simulink model "drive_fb_pack"  (R2026b)
settings: Solver=VariableStepAuto
undefined symbols (not defined in the file or in its folder): P
libraries: svdutilitieslib x3
settings Model: Creator=aomar  LastModifiedBy=aomar

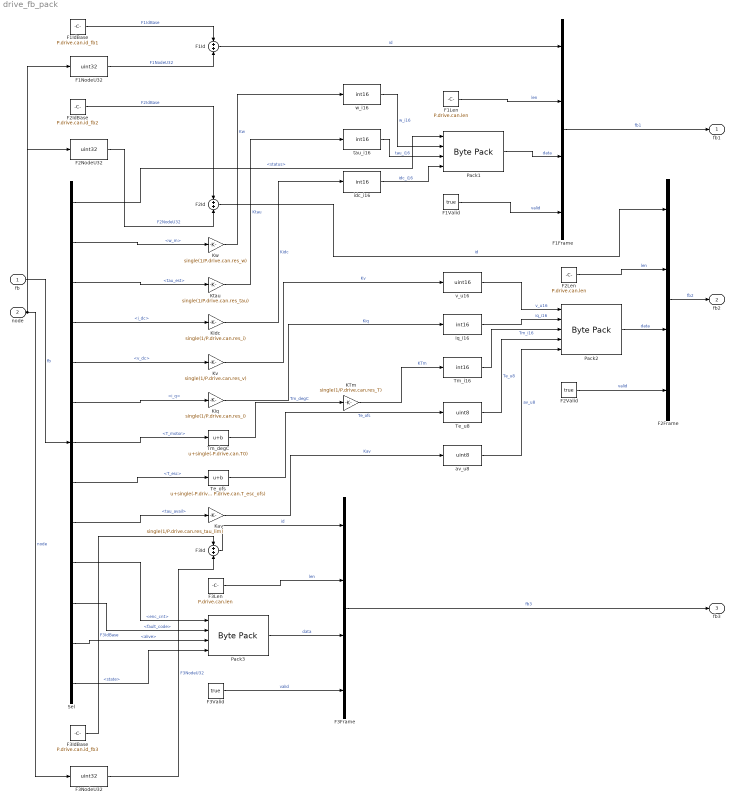
== system drive_fb_pack ==
  fb : Inport  OutDataTypeStr=Bus: Bus_DriveSideFb
  node : Inport  Port=2  OutDataTypeStr=uint8
  F1Frame : BusCreator  Inputs=4  OutDataTypeStr=Bus: Bus_CanFrame8  NonVirtualBus=on
  F1Id : Sum  OutDataTypeStr=uint32  SaturateOnIntegerOverflow=on
  F1IdBase : Constant  Value=P.drive.can.id_fb1  OutDataTypeStr=uint32
  F1Len : Constant  Value=P.drive.can.len  OutDataTypeStr=uint8
  F1NodeU32 : DataTypeConversion  OutDataTypeStr=uint32  RndMeth=Nearest
  F1Valid : Constant  Value=true  OutDataTypeStr=boolean
  F2Frame : BusCreator  Inputs=4  OutDataTypeStr=Bus: Bus_CanFrame8  NonVirtualBus=on
  F2Id : Sum  OutDataTypeStr=uint32  SaturateOnIntegerOverflow=on
  F2IdBase : Constant  Value=P.drive.can.id_fb2  OutDataTypeStr=uint32
  F2Len : Constant  Value=P.drive.can.len  OutDataTypeStr=uint8
  F2NodeU32 : DataTypeConversion  OutDataTypeStr=uint32  RndMeth=Nearest
  F2Valid : Constant  Value=true  OutDataTypeStr=boolean
  F3Frame : BusCreator  Inputs=4  OutDataTypeStr=Bus: Bus_CanFrame8  NonVirtualBus=on
  F3Id : Sum  OutDataTypeStr=uint32  SaturateOnIntegerOverflow=on
  F3IdBase : Constant  Value=P.drive.can.id_fb3  OutDataTypeStr=uint32
  F3Len : Constant  Value=P.drive.can.len  OutDataTypeStr=uint8
  F3NodeU32 : DataTypeConversion  OutDataTypeStr=uint32  RndMeth=Nearest
  F3Valid : Constant  Value=true  OutDataTypeStr=boolean
  KTm : Gain  Gain=single(1/P.drive.can.res_T)
  Kav : Gain  Gain=single(1/P.drive.can.res_tau_lim)
  Kidc : Gain  Gain=single(1/P.drive.can.res_i)
  Kiq : Gain  Gain=single(1/P.drive.can.res_i)
  Ktau : Gain  Gain=single(1/P.drive.can.res_tau)
  Kv : Gain  Gain=single(1/P.drive.can.res_v)
  Kw : Gain  Gain=single(1/P.drive.can.res_w)
  Pack1 : svdutilitieslib/Byte Pack  maskPackedDataType=uint8  datatypes={'uint16','int16','int16','int16'}  byteAlign=1  blockPlatform=arduinoert
      settings: LibrarySourceBlock=mcblib/Signal Management/Byte Pack
  Pack2 : svdutilitieslib/Byte Pack  maskPackedDataType=uint8  datatypes={'uint16','int16','int16','uint8','uint8'}  byteAlign=1  blockPlatform=arduinoert
      settings: LibrarySourceBlock=mcblib/Signal Management/Byte Pack
  Pack3 : svdutilitieslib/Byte Pack  maskPackedDataType=uint8  datatypes={'int32','uint16','uint8','uint8'}  byteAlign=1  blockPlatform=arduinoert
      settings: LibrarySourceBlock=mcblib/Signal Management/Byte Pack
  Sel : BusSelector  OutputSignals=status,w_m,tau_est,i_dc,v_dc,i_q,T_motor,T_esc,tau_avail,enc_cnt,fault_code,alive,state
  Te_ofs : Bias  Bias=single(-P.drive.can.T0 + P.drive.can.T_esc_ofs)  SaturateOnIntegerOverflow=off
  Te_u8 : DataTypeConversion  OutDataTypeStr=uint8  RndMeth=Nearest
  Tm_degC : Bias  Bias=single(-P.drive.can.T0)  SaturateOnIntegerOverflow=off
  Tm_i16 : DataTypeConversion  OutDataTypeStr=int16  RndMeth=Nearest
  av_u8 : DataTypeConversion  OutDataTypeStr=uint8  RndMeth=Nearest
  idc_i16 : DataTypeConversion  OutDataTypeStr=int16  RndMeth=Nearest
  iq_i16 : DataTypeConversion  OutDataTypeStr=int16  RndMeth=Nearest
  tau_i16 : DataTypeConversion  OutDataTypeStr=int16  RndMeth=Nearest
  v_u16 : DataTypeConversion  OutDataTypeStr=uint16  RndMeth=Nearest
  w_i16 : DataTypeConversion  OutDataTypeStr=int16  RndMeth=Nearest
  fb1 : Outport  OutDataTypeStr=Bus: Bus_CanFrame8
  fb2 : Outport  Port=2  OutDataTypeStr=Bus: Bus_CanFrame8
  fb3 : Outport  Port=3  OutDataTypeStr=Bus: Bus_CanFrame8
  wires:
  fb/1 -> Sel/1  "fb"
  node/1 -> F3NodeU32/1, F1NodeU32/1, F2NodeU32/1  "node"
  Sel/1 -> Pack1/1  "<status>"
  Sel/2 -> Kw/1  "<w_m>"
  Sel/3 -> Ktau/1  "<tau_est>"
  Sel/4 -> Kidc/1  "<i_dc>"
  Sel/5 -> Kv/1  "<v_dc>"
  Sel/6 -> Kiq/1  "<i_q>"
  Sel/7 -> Tm_degC/1  "<T_motor>"
  Sel/8 -> Te_ofs/1  "<T_esc>"
  Sel/9 -> Kav/1  "<tau_avail>"
  Sel/10 -> Pack3/1  "<enc_cnt>"
  Sel/11 -> Pack3/2  "<fault_code>"
  Sel/12 -> Pack3/3  "<alive>"
  Sel/13 -> Pack3/4  "<state>"
  F1IdBase/1 -> F1Id/1  "F1IdBase"
  F2IdBase/1 -> F2Id/1  "F2IdBase"
  F3IdBase/1 -> F3Id/1  "F3IdBase"
  F1NodeU32/1 -> F1Id/2  "F1NodeU32"
  F2NodeU32/1 -> F2Id/2  "F2NodeU32"
  F3NodeU32/1 -> F3Id/2  "F3NodeU32"
  F1Id/1 -> F1Frame/1  "id"
  F2Id/1 -> F2Frame/1  "id"
  F3Id/1 -> F3Frame/1  "id"
  Kw/1 -> w_i16/1  "Kw"
  Ktau/1 -> tau_i16/1  "Ktau"
  Kidc/1 -> idc_i16/1  "Kidc"
  Kv/1 -> v_u16/1  "Kv"
  Kiq/1 -> iq_i16/1  "Kiq"
  Kav/1 -> av_u8/1  "Kav"
  F3Len/1 -> F3Frame/2  "len"
  F3Valid/1 -> F3Frame/4  "valid"
  Tm_degC/1 -> KTm/1  "Tm_degC"
  Te_ofs/1 -> Te_u8/1  "Te_ofs"
  Pack3/1 -> F3Frame/3  "data"
  F3Frame/1 -> fb3/1  "fb3"
  KTm/1 -> Tm_i16/1  "KTm"
  w_i16/1 -> Pack1/2  "w_i16"
  tau_i16/1 -> Pack1/3  "tau_i16"
  idc_i16/1 -> Pack1/4  "idc_i16"
  F1Len/1 -> F1Frame/2  "len"
  F1Valid/1 -> F1Frame/4  "valid"
  v_u16/1 -> Pack2/1  "v_u16"
  iq_i16/1 -> Pack2/2  "iq_i16"
  Tm_i16/1 -> Pack2/3  "Tm_i16"
  Te_u8/1 -> Pack2/4  "Te_u8"
  av_u8/1 -> Pack2/5  "av_u8"
  Pack1/1 -> F1Frame/3  "data"
  F1Frame/1 -> fb1/1  "fb1"
  F2Len/1 -> F2Frame/2  "len"
  F2Valid/1 -> F2Frame/4  "valid"
  Pack2/1 -> F2Frame/3  "data"
  F2Frame/1 -> fb2/1  "fb2"
